simulink library "Lib_Piccolo"  (R2018b)
settings: Solver=VariableStepAuto  StartTime=0.0  StopTime=10.0  RelTol=1e-3
values from neighbouring files (symbols this model uses):
  AccelErrInt2Brakes = 0.15    [SimulationControlConfig16P.m]    (also in SimulationControlConfig16P_LEGACY.m; SimulationControlConfigTAILLESS.m = 0.2; SimulationControlConfigUTAIL.m = 0.2)
  AileronMax = 25    [SimulationControlConfig16P.m]    (also in SimulationControlConfig16P_LEGACY.m; SimulationControlConfigTAILLESS.m; SimulationControlConfigUTAIL.m)
  AileronPower = 0.00268    [SimulationControlConfig16P.m]    (also in SimulationControlConfig16P_LEGACY.m; SimulationControlConfigTAILLESS.m; SimulationControlConfigUTAIL.m)
  AileronSurfaceMax = 45    [SimulationControlConfig16P.m]    (also in SimulationControlConfig16P_LEGACY.m)
  AileronTrim = 0    [SimulationControlConfig16P.m]    (also in SimulationControlConfig16P_LEGACY.m; SimulationControlConfigTAILLESS.m; SimulationControlConfigUTAIL.m)
  Alt = 1000 + TerrainHeight    [SimulationStateConfig.m]
  AltCruise_m = testPlans(testIndx).terrainElevation * 0.3048 + 200    [SimulationControlConfig16P.m]    (also in SimulationControlConfigTAILLESS.m = 1083; SimulationControlConfigUTAIL.m = testPlans(testIndx).terrainElevation * 0.3048 + 152)
  AltitudeRate2PitchCmdIntegratorInit = 0.1    [SimulationControlPre.m]
  AltMax = 10000    [SimulationControlConfig16P.m]    (also in SimulationControlConfig16P_LEGACY.m; SimulationControlConfigTAILLESS.m; SimulationControlConfigUTAIL.m)
  AltMaxAccel = 1.25    [SimulationControlConfig16P.m]    (also in SimulationControlConfig16P_LEGACY.m = 0.9; SimulationControlConfigTAILLESS.m = 1.7; SimulationControlConfigUTAIL.m = 2)
  AltMin = 0    [SimulationControlConfig16P.m]    (also in SimulationControlConfig16P_LEGACY.m; SimulationControlConfigTAILLESS.m; SimulationControlConfigUTAIL.m)
  AltRateCmd2Pitch = 0.50    (= 0.5)    [SimulationControlConfig16P.m]    (also in SimulationControlConfig16P_LEGACY.m = 0.6; SimulationControlConfigTAILLESS.m = 0.2; SimulationControlConfigUTAIL.m = 0.3)
  AltRateError2Pitch = 0.40    (= 0.4)    [SimulationControlConfig16P.m]    (also in SimulationControlConfig16P_LEGACY.m; SimulationControlConfigTAILLESS.m = 0.55; SimulationControlConfigUTAIL.m = 0.55)
  AltRateErrorInt2Pitch = 0.50    (= 0.5)    [SimulationControlConfig16P.m]    (also in SimulationControlConfig16P_LEGACY.m = 0.45; SimulationControlConfigTAILLESS.m; SimulationControlConfigUTAIL.m = 0.75)
  AltRateLpfCutOff = 3    [SimulationControlConfig16P.m]    (also in SimulationControlConfig16P_LEGACY.m; SimulationControlConfigTAILLESS.m = 2; SimulationControlConfigUTAIL.m = 2)
  AutoNosegear2Rudder = 26    [SimulationControlConfig16P.m]    (also in SimulationControlConfig16P_LEGACY.m; SimulationControlConfigTAILLESS.m = 25.2; SimulationControlConfigUTAIL.m = 14)
  b = 5.54    [SimulationControlConfig16P.m]    (also in SimulationControlConfig16P_LEGACY.m; SimulationControlConfigTAILLESS.m = 2.37; SimulationControlConfigUTAIL.m = 2.37)
  Bank2AileronIntegratorInit = 0    [SimulationControlPre.m]
  BankMax_User = BankMax_User/180*pi    (= 0.523598775598)    [SimulationControlConfig16P.m]    (also in SimulationControlConfig16P_LEGACY.m; SimulationControlConfigTAILLESS.m = 0.610865238198; SimulationControlConfigUTAIL.m = 0.628318530718)
  baseLegFlaps = 20    [SimulationControlConfig16P.m]    (also in SimulationControlConfig16P_LEGACY.m = 0; SimulationControlConfigTAILLESS.m = 15; SimulationControlConfigUTAIL.m = 10)
  C = GeneticOpt.C    [SimulationCostFunction.m]
  c = Sw/b    (= 0.841696750903)    [SimulationControlConfig16P.m]    (also in SimulationControlConfig16P_LEGACY.m; SimulationControlConfigTAILLESS.m = 0.354008438819; SimulationControlConfigUTAIL.m = 0.354008438819)
  cell2WheelFactorMG = 5.98    [SimulationSensorConfig16P_LEGACY.m]
  cell2WheelFactorNG = 1    [SimulationSensorConfig16P_LEGACY.m]
  cellSatMaxMG = 15000    [SimulationSensorConfig16P.m]    (also in SimulationSensorConfig16P_LEGACY.m; SimulationSensorConfigTAILLESS7P.m; SimulationSensorConfigUTAIL7P.m)
  cellSatMaxNG = 1000    [SimulationSensorConfig16P.m]    (also in SimulationSensorConfig16P_LEGACY.m; SimulationSensorConfigTAILLESS7P.m; SimulationSensorConfigUTAIL7P.m)
  cellSatMinMG = -15000    [SimulationSensorConfig16P.m]    (also in SimulationSensorConfig16P_LEGACY.m; SimulationSensorConfigTAILLESS7P.m; SimulationSensorConfigUTAIL7P.m)
  cellSatMinNG = -1000    [SimulationSensorConfig16P.m]    (also in SimulationSensorConfig16P_LEGACY.m; SimulationSensorConfigTAILLESS7P.m; SimulationSensorConfigUTAIL7P.m)
  CL_Limit = CL_Max    (= 0.54)    [SimulationControlConfig16P.m]    (also in SimulationControlConfig16P_LEGACY.m; SimulationControlConfigTAILLESS.m; SimulationControlConfigUTAIL.m = 0.53)
  CL_Max = 0.54    [SimulationControlConfig16P.m]    (also in SimulationControlConfig16P_LEGACY.m; SimulationControlConfigTAILLESS.m; SimulationControlConfigUTAIL.m = 0.53)
  CL_Max_Nom = 0.465    [SimulationControlConfig16P.m]    (also in SimulationControlConfig16P_LEGACY.m; SimulationControlConfigTAILLESS.m = 0.39; SimulationControlConfigUTAIL.m)
  CL_Min = 0    [SimulationControlConfig16P.m]    (also in SimulationControlConfig16P_LEGACY.m; SimulationControlConfigTAILLESS.m; SimulationControlConfigUTAIL.m)
  ClimbMaxFraction = 0.35    [SimulationControlConfig16P.m]    (also in SimulationControlConfig16P_LEGACY.m = 0.24; SimulationControlConfigTAILLESS.m = 0.19; SimulationControlConfigUTAIL.m = 0.21)
  ClimboutMaxBank = 7.0    (= 7)    [SimulationControlConfig16P.m]    (also in SimulationControlConfig16P_LEGACY.m; SimulationControlConfigTAILLESS.m = 5; SimulationControlConfigUTAIL.m)
  ClimboutTimer = 7.0    (= 7)    [SimulationControlConfig16P.m]    (also in SimulationControlConfig16P_LEGACY.m; SimulationControlConfigTAILLESS.m; SimulationControlConfigUTAIL.m)
  dCl_per_dFlap = 0.005581818    [SimulationControlConfig16P.m]    (also in SimulationControlConfig16P_LEGACY.m = 0; SimulationControlConfigTAILLESS.m = 0; SimulationControlConfigUTAIL.m = 0)
  DecelerationCmd = 3.1    [SimulationControlConfig16P.m]    (also in SimulationControlConfig16P_LEGACY.m; SimulationControlConfigTAILLESS.m = 0.1; SimulationControlConfigUTAIL.m = 0.1)
  DeRotateLogicEndTimer = abs((NoseDownLimit_Deg-1)/DeRotateRamp_Dps)    [SimulationControlConfig16P.m]    (also in SimulationControlConfig16P_LEGACY.m; SimulationControlConfigTAILLESS.m; SimulationControlConfigUTAIL.m)
  DeRotateLogicHoldNoseUpTimer = 0.1    [SimulationControlConfig16P.m]    (also in SimulationControlConfig16P_LEGACY.m; SimulationControlConfigTAILLESS.m; SimulationControlConfigUTAIL.m)
  DeRotateLogicTimerTimeout = 2    [SimulationControlConfig16P.m]    (also in SimulationControlConfig16P_LEGACY.m; SimulationControlConfigTAILLESS.m; SimulationControlConfigUTAIL.m)
  DeRotateLowerCmdSaturation = 0    [SimulationControlConfig16P.m]    (also in SimulationControlConfig16P_LEGACY.m; SimulationControlConfigTAILLESS.m; SimulationControlConfigUTAIL.m)
  DeRotateRamp_Dps = 3    [SimulationControlConfig16P.m]    (also in SimulationControlConfig16P_LEGACY.m; SimulationControlConfigTAILLESS.m = 8; SimulationControlConfigUTAIL.m = 8)
  DeRotateUpperCmdSaturation = 7    [SimulationControlConfig16P.m]    (also in SimulationControlConfig16P_LEGACY.m; SimulationControlConfigTAILLESS.m; SimulationControlConfigUTAIL.m)
  DescentMaxFraction = 0.22    [SimulationControlConfig16P.m]    (also in SimulationControlConfig16P_LEGACY.m = 0.2; SimulationControlConfigTAILLESS.m = 0.17; SimulationControlConfigUTAIL.m = 0.17)
  DesktopSimTerrainOffset_m = 0.406    [SimulationAircraftConfig.m]
  downwindFlaps = 0    [SimulationControlConfig16P.m]    (also in SimulationControlConfig16P_LEGACY.m; SimulationControlConfigTAILLESS.m; SimulationControlConfigUTAIL.m)
  DP_init = 0.5*1.225*V_init^2    [SimulationControlConfig16P.m]    (also in SimulationControlConfig16P_LEGACY.m; SimulationControlConfigTAILLESS.m; SimulationControlConfigUTAIL.m)
  dscNoiseMG = 1    [SimulationSensorConfig16P_LEGACY.m]
  dscNoiseNG = 0.25    [SimulationSensorConfig16P_LEGACY.m]
  DSCnumBits = 24    [SimulationSensorConfig16P.m]    (also in SimulationSensorConfig16P_LEGACY.m; SimulationSensorConfigTAILLESS7P.m; SimulationSensorConfigUTAIL7P.m)
  DSCRangeMaxMG = 15000    [SimulationSensorConfig16P.m]    (also in SimulationSensorConfig16P_LEGACY.m; SimulationSensorConfigTAILLESS7P.m; SimulationSensorConfigUTAIL7P.m)
  DSCRangeMaxNG = 1000    [SimulationSensorConfig16P.m]    (also in SimulationSensorConfig16P_LEGACY.m; SimulationSensorConfigTAILLESS7P.m; SimulationSensorConfigUTAIL7P.m)
  DSCRangeMinMG = -15000    [SimulationSensorConfig16P.m]    (also in SimulationSensorConfig16P_LEGACY.m; SimulationSensorConfigTAILLESS7P.m; SimulationSensorConfigUTAIL7P.m)
  DSCRangeMinNG = -1000    [SimulationSensorConfig16P.m]    (also in SimulationSensorConfig16P_LEGACY.m; SimulationSensorConfigTAILLESS7P.m; SimulationSensorConfigUTAIL7P.m)
  dt = DLLSim.dt    [SimulationTimeStep.m]    (also in SimulationTrim.m = 0.02)
  EarlyTouchdownThreshold = 3.0    (= 3)    [SimulationControlConfig16P.m]    (also in SimulationControlConfig16P_LEGACY.m; SimulationControlConfigTAILLESS.m = 2.2; SimulationControlConfigUTAIL.m = 2.5)
  ElevatorDeflectionRate = 15    [SimulationControlConfig16P.m]    (also in SimulationControlConfig16P_LEGACY.m = 12; SimulationControlConfigTAILLESS.m = 10; SimulationControlConfigUTAIL.m = 12)
  ElevatorMax = 25    [SimulationControlConfig16P.m]    (also in SimulationControlConfig16P_LEGACY.m; SimulationControlConfigTAILLESS.m; SimulationControlConfigUTAIL.m)
  ElevatorPower = -0.002209    [SimulationControlConfig16P.m]    (also in SimulationControlConfig16P_LEGACY.m; SimulationControlConfigTAILLESS.m = -0.002956; SimulationControlConfigUTAIL.m = -0.00205983)
  ElevatorTrim = -3.5    [SimulationControlConfig16P.m]    (also in SimulationControlConfig16P_LEGACY.m; SimulationControlConfigTAILLESS.m = -6; SimulationControlConfigUTAIL.m = -8)
  elevonBias = 0    [SimulationControlConfig16P.m]    (also in SimulationControlConfig16P_LEGACY.m; SimulationControlConfigTAILLESS.m; SimulationControlConfigUTAIL.m)
  Enable_TAS_Protection = 0    [SimulationControlConfig16P.m]    (also in SimulationControlConfig16P_LEGACY.m; SimulationControlConfigTAILLESS.m; SimulationControlConfigUTAIL.m)
  EnableCrossTrackAbort = 1    [SimulationControlConfig16P.m]    (also in SimulationControlConfigTAILLESS.m; SimulationControlConfigUTAIL.m)
  EnergyBandwidth = 0.02    [SimulationControlConfig16P.m]    (also in SimulationControlConfig16P_LEGACY.m; SimulationControlConfigTAILLESS.m = 0.06; SimulationControlConfigUTAIL.m = 0.06)
  EngineLhFuelCut = 0    [SimulationAircraftConfig.m]
  EngineRhFuelCut = 0    [SimulationAircraftConfig.m]
  FastThrottleRate = 0.075    [SimulationControlConfig16P.m]    (also in SimulationControlConfig16P_LEGACY.m = 0.05; SimulationControlConfigTAILLESS.m = 0.1; SimulationControlConfigUTAIL.m = 0.1)
  FilterWarmUpTime = 2    [SimulationSensorConfig16P.m]    (also in SimulationSensorConfig16P_LEGACY.m; SimulationSensorConfigTAILLESS7P.m; SimulationSensorConfigUTAIL7P.m)
  finalApproachFlaps = 20    [SimulationControlConfig16P.m]    (also in SimulationControlConfig16P_LEGACY.m = 0; SimulationControlConfigTAILLESS.m = 22; SimulationControlConfigUTAIL.m = 10)
  FinalDescentSlope_Deg = testPlans(testIndx).descentSlope    [SimulationControlConfig16P.m]    (also in SimulationControlConfig16P_LEGACY.m; SimulationControlConfigTAILLESS.m; SimulationControlConfigUTAIL.m)
  flapMax = 0    [SimulationControlConfig16P.m]    (also in SimulationControlConfig16P_LEGACY.m; SimulationControlConfigTAILLESS.m; SimulationControlConfigUTAIL.m)
  flapRate = 7.5    [SimulationControlConfig16P.m]    (also in SimulationControlConfig16P_LEGACY.m; SimulationControlConfigTAILLESS.m = 6.6; SimulationControlConfigUTAIL.m)
  FlareHeight = 5    [SimulationControlConfig16P.m]    (also in SimulationControlConfig16P_LEGACY.m = 4.8; SimulationControlConfigTAILLESS.m = 2.5; SimulationControlConfigUTAIL.m = 2)
  FlareVerticalRate_mps = -0.4    [SimulationControlConfig16P.m]    (also in SimulationControlConfig16P_LEGACY.m = -0.5; SimulationControlConfigTAILLESS.m = -0.15; SimulationControlConfigUTAIL.m = -0.15)
  Fp_Aileron = 0.55*2*pi*RollRateLpfCutoff*dt    [SimulationControlConfig16P.m]    (also in SimulationControlConfig16P_LEGACY.m; SimulationControlConfigTAILLESS.m; SimulationControlConfigUTAIL.m)
  Fp_Alt = 0.55*AltBandwidth    (= 0.099)    [SimulationControlConfig16P.m]    (also in SimulationControlConfig16P_LEGACY.m; SimulationControlConfigTAILLESS.m = 0.587477826221; SimulationControlConfigUTAIL.m = 0.69115038379)
  Fp_AltRate = 0.55*2*pi*AltRateLpfCutOff*dt    [SimulationControlConfig16P.m]    (also in SimulationControlConfig16P_LEGACY.m; SimulationControlConfigTAILLESS.m; SimulationControlConfigUTAIL.m)
  Fp_Elevator = 0.55*2*pi*PitchRateLpfCutoff*dt    [SimulationControlConfig16P.m]    (also in SimulationControlConfig16P_LEGACY.m; SimulationControlConfigTAILLESS.m; SimulationControlConfigUTAIL.m)
  Fp_Energy = 0.55*2*pi*EnergyBandwidth    (= 0.069115038379)    [SimulationControlConfig16P.m]    (also in SimulationControlConfig16P_LEGACY.m; SimulationControlConfigTAILLESS.m = 0.207345115137; SimulationControlConfigUTAIL.m = 0.207345115137)
  Fp_Energy2 = 0.55*2*pi*EnergyBandwidth*dt    [SimulationControlConfig16P.m]    (also in SimulationControlConfig16P_LEGACY.m; SimulationControlConfigTAILLESS.m; SimulationControlConfigUTAIL.m)
  Fp_Pitch = 0.55*2*pi*PitchBandwidth    (= 2.76460153516)    [SimulationControlConfig16P.m]    (also in SimulationControlConfig16P_LEGACY.m = 3.11017672705; SimulationControlConfigTAILLESS.m = 3.80132711084; SimulationControlConfigUTAIL.m = 2.41902634326)
  Fp_Pitch_2 = 0.55*2*pi*PitchBandwidth*dt    [SimulationControlConfig16P.m]    (also in SimulationControlConfig16P_LEGACY.m; SimulationControlConfigTAILLESS.m; SimulationControlConfigUTAIL.m)
  Fp_Roll = RollBandwidth^2    (= 1)    [SimulationControlConfig16P.m]    (also in SimulationControlConfig16P_LEGACY.m = 1.44; SimulationControlConfigTAILLESS.m; SimulationControlConfigUTAIL.m)
  Fp_Rudder = 0.55*2*pi*YawRateLpfCutoff*dt    [SimulationControlConfig16P.m]    (also in SimulationControlConfig16P_LEGACY.m; SimulationControlConfigTAILLESS.m; SimulationControlConfigUTAIL.m)
  Fp_TAS = 0.55*2*pi*TASBandwidth    (= 0.103672557568)    [SimulationControlConfig16P.m]    (also in SimulationControlConfig16P_LEGACY.m; SimulationControlConfigTAILLESS.m = 0.172787595947; SimulationControlConfigUTAIL.m = 0.172787595947)
  Fp_TAS_Filter = 2*pi*TasLpfCutoff*dt    [SimulationControlConfig16P.m]    (also in SimulationControlConfig16P_LEGACY.m; SimulationControlConfigTAILLESS.m; SimulationControlConfigUTAIL.m)
  Fp_Turn = 0.55*2*pi*TurnErrLPFcutoff    (= 0.0345575191895)    [SimulationControlConfig16P.m]    (also in SimulationControlConfig16P_LEGACY.m; SimulationControlConfigTAILLESS.m = 0.172787595947; SimulationControlConfigUTAIL.m = 0.172787595947)
  Fp_TurnDerr = 0.55*2*pi*TurnDerivativeLPFcutoff    (= 0.0345575191895)    [SimulationControlConfig16P.m]    (also in SimulationControlConfig16P_LEGACY.m; SimulationControlConfigTAILLESS.m = 0.172787595947; SimulationControlConfigUTAIL.m = 0.172787595947)
  FTV = 3    [SimulationAircraftConfig.m]
  ftvStaticPositionError = 1/1.18    (= 0.847457627119)    [SimulationSensorConfig16P.m]    (also in SimulationSensorConfig16P_LEGACY.m; SimulationSensorConfigTAILLESS7P.m = 1; SimulationSensorConfigUTAIL7P.m = 1)
  g = 9.81    [SimulationStateConfig.m]
  GustSpd_Kts = testPlans(testIndx).gustSpd    [SimulationStateConfig.m]
  GustTriggerVal = testPlans(testIndx).gustTriggerVal    [SimulationStateConfig.m]
  HeadingErr2TurnRate = 0.5    [SimulationControlConfig16P.m]    (also in SimulationControlConfig16P_LEGACY.m; SimulationControlConfigTAILLESS.m; SimulationControlConfigUTAIL.m)
  HeadingErrDer2TurnRate = 0.3    [SimulationControlConfig16P.m]    (also in SimulationControlConfig16P_LEGACY.m; SimulationControlConfigTAILLESS.m; SimulationControlConfigUTAIL.m)
  IASbounce = IASstall*0.8    [SimulationControlPre.m]
  IAScruiseCMD = sqrt(2*m*9.81/(1.225*Sw*CL_cruise))    [SimulationControlConfig16P.m]    (also in SimulationControlConfig16P_LEGACY.m; SimulationControlConfigTAILLESS.m; SimulationControlConfigUTAIL.m)
  IASfinalCMD = 1.12 * IASmin    [SimulationControlConfig16P.m]    (also in SimulationControlConfig16P_LEGACY.m = 1.10 * IASmin; SimulationControlConfigTAILLESS.m = 1.10 * IASmin; SimulationControlConfigUTAIL.m = 1.15 * IASmin)
  IASflareCMD = IASstall    [SimulationControlConfig16P.m]    (also in SimulationControlConfig16P_LEGACY.m; SimulationControlConfigTAILLESS.m; SimulationControlConfigUTAIL.m)
  IASmax = 64    [SimulationControlConfig16P.m]    (also in SimulationControlConfig16P_LEGACY.m = 46; SimulationControlConfigTAILLESS.m = 38.58; SimulationControlConfigUTAIL.m = 35)
  IASmin = sqrt(2*m*9.81/(1.225*Sw*0.9*CL_Max_Nom))    [SimulationControlConfig16P.m]    (also in SimulationControlConfig16P_LEGACY.m; SimulationControlConfigTAILLESS.m; SimulationControlConfigUTAIL.m)
  IASshortCMD = IASstall    [SimulationControlConfig16P.m]    (also in SimulationControlConfig16P_LEGACY.m; SimulationControlConfigTAILLESS.m; SimulationControlConfigUTAIL.m)
  IASstall = sqrt(2*m*9.81/(1.225*Sw*CL_Max))    [SimulationControlConfig16P.m]    (also in SimulationControlConfig16P_LEGACY.m; SimulationControlConfigTAILLESS.m; SimulationControlConfigUTAIL.m)
  inFlight = 1    [SimulationControlConfig16P.m]    (also in SimulationControlConfigTAILLESS.m; SimulationControlConfigUTAIL.m)
  JetCatOffset = 5    [SimulationControlConfig16P.m]    (also in SimulationControlConfig16P_LEGACY.m)
  LaunchRollingElevator = -1.5    [SimulationControlConfig16P.m]    (also in SimulationControlConfig16P_LEGACY.m; SimulationControlConfigTAILLESS.m = 1; SimulationControlConfigUTAIL.m = 1)
  ldg_NosegearMax = 10    [SimulationControlConfig16P.m]    (also in SimulationControlConfig16P_LEGACY.m; SimulationControlConfigTAILLESS.m; SimulationControlConfigUTAIL.m)
  ldg_TrackVyErrInt2Nosegear = 0.1250    (= 0.125)    [SimulationControlConfig16P.m]    (also in SimulationControlConfig16P_LEGACY.m; SimulationControlConfigTAILLESS.m = 0.00714285714286; SimulationControlConfigUTAIL.m = 0.00714285714286)
  ldg_TrackVyErrPro2Nosegear = 0.35    [SimulationControlConfig16P.m]    (also in SimulationControlConfig16P_LEGACY.m; SimulationControlConfigTAILLESS.m = 0.0546666666667; SimulationControlConfigUTAIL.m = 0.0546666666667)
  ldg_TrackY2Vy = 0.07    [SimulationControlConfig16P.m]    (also in SimulationControlConfig16P_LEGACY.m; SimulationControlConfigTAILLESS.m = 0.17; SimulationControlConfigUTAIL.m = 0.17)
  ldg_Vy2NosegearScalingPower = 1.075    [SimulationControlConfig16P.m]    (also in SimulationControlConfig16P_LEGACY.m; SimulationControlConfigTAILLESS.m = 0.6; SimulationControlConfigUTAIL.m = 0.5)
  ldg_Y2VyScalingPower = 0.175    [SimulationControlConfig16P.m]    (also in SimulationControlConfig16P_LEGACY.m; SimulationControlConfigTAILLESS.m = 0; SimulationControlConfigUTAIL.m = 0)
  ldg_YawRate2Nosegear = 0.175    [SimulationControlConfig16P.m]    (also in SimulationControlConfig16P_LEGACY.m; SimulationControlConfigTAILLESS.m = 0.065; SimulationControlConfigUTAIL.m = 0.065)
  LiftSlope = 0.064285    [SimulationControlConfig16P.m]    (also in SimulationControlConfig16P_LEGACY.m; SimulationControlConfigTAILLESS.m = 0.058631; SimulationControlConfigUTAIL.m)
  LPFaileronInit = 0    [SimulationControlPre.m]
  LPFclestInit = 0    [SimulationControlPre.m]
  LPFenergyFFInit = 0    [SimulationControlPre.m]
  LPFtasInit = V_init + 2    [SimulationControlPre.m]
  LPFthrottleInit = ThrottleTrim    [SimulationControlPre.m]
  LPFturnErrInit = 0    [SimulationControlPre.m]
  ... (+115 more)
undefined symbols (not defined in the file or in its folder): abortFlag, alphaHPF, apmDelay, BRWNOUT, CRAWOR, CRAWUR, DiscIntNeverNeededParam, DLLSim, DLLSimStep, ECOMOR, ECOMUR, Fp_Tas, GustTrigger_HeightAgl_m, IPSTAT, LCINTEG, Ldg_Persist_Time, LOWER_FLAGS, MSG_ENABLE, NoiseStd, OLDVAL, OVERRIDE_ENABLE, OVERRIDE_VALUE, REBOOT, reversionEnable, revIASMax, revIASMin, revPitchMax, revPitchMin, revPitchRateMax, revRollMax, revRollRateMax, SAMPLE, SCALON, SensorModel, sigbuilder_block, Sim_Vx, Sim_Vy, Sim_Vz, Sim_Xpos, Sim_Ypos, Sim_Zpos, SYSOR, SYSUR, TARE, TEMPOR, TEMPUR, testIndx, testPlan, testPlans, Trim_piccoloInCmd, Trim_REFSI_FD_IN_nmodeCgShifterCmd_Ft, Trim_REFSI_FD_IN_nmodeFlapLhIBCmd_Deg, Trim_REFSI_FD_IN_nmodeFlapLhOBCmd_Deg, Trim_REFSI_FD_IN_nmodeFlapRhIBCmd_Deg, Trim_REFSI_FD_IN_nmodeFlapRhOBCmd_Deg, Trim_REFSI_FD_IN_nmodeSlatLhCmd_Deg, Trim_REFSI_FD_IN_nmodeSlatRhCmd_Deg, Trim_REFSI_FD_IN_nmodeSplrLhInbdCmd_Deg, Trim_REFSI_FD_IN_nmodeSplrLhOutbdCmd_Deg ... (+5)
libraries: simulink x866, aerolibconvert2 x60, $bdroot x52, aerolibatmos2 x5, dspswit3 x5, simulink_extras x4, dsparch4 x2, Lib_Piccolo_Alt x2, eeGeneralControl x1, dspindex x1
(part 1 of 44)
settings Model: Creator=ghoward  LastModifiedBy=JFigueira-Admin

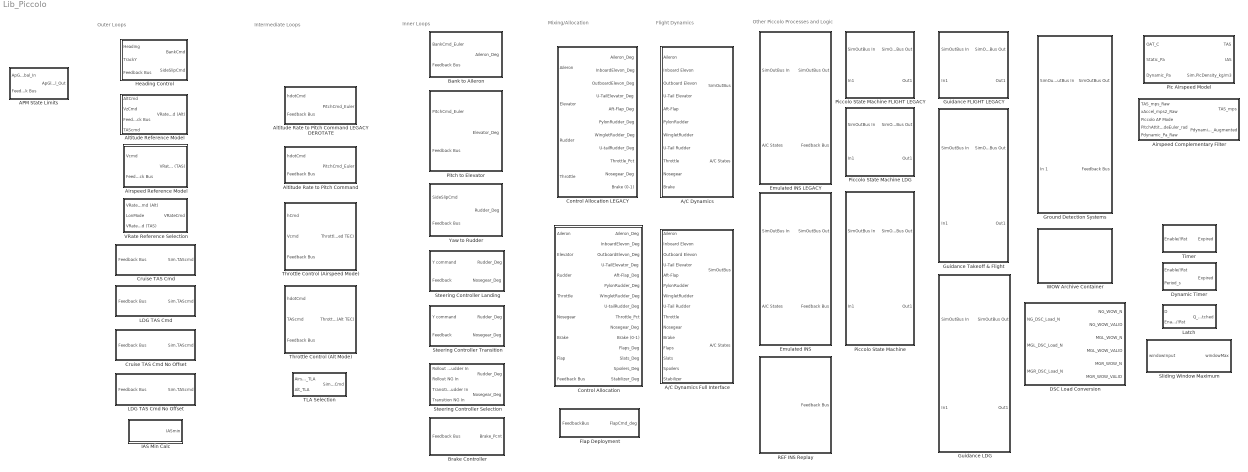
== system Lib_Piccolo ==
  note: Inner Loops
  note: Outer Loops
  note: Intermediate Loops
  note: Mixing/Allocation
  note: Other Piccolo Processes and Logic
  note: Flight Dynamics
  " Dynamic Timer" : Subsystem
      mask DialogControl DescTextVar Prompt: Timer with variable period provided as an input. Period will only be updated when reset (!RST) is active.
  " Timer" : Subsystem  mask{period=Ldg_Persist_Time}
      mask prompts: period "Period [s]"
      mask DialogControl DescGroupVar Prompt: Timer
      mask DialogControl DescTextVar Prompt: A basic timer with period as defined in mask
  A/C Dynamics : Subsystem
  A/C Dynamics Full Interface : Subsystem
  APM State Limits : Subsystem
  Airspeed Complementary Filter : Subsystem
  Airspeed Reference Model : Subsystem
  Altitude Rate to Pitch Command : Subsystem
  Altitude Rate to Pitch Command LEGACY DEROTATE : Subsystem
  Altitude Reference Model : Subsystem
  Bank to Aileron : Subsystem
  Brake Controller : Subsystem
  Control Allocation : Subsystem  Variant=on
  Control Allocation LEGACY : Subsystem
  Cruise TAS Cmd : Subsystem
  Cruise TAS Cmd No Offset : Subsystem
  DSC Load Conversion : Subsystem
  Emulated INS : Subsystem
  Emulated INS LEGACY : Subsystem
  Flap Deployment : Subsystem
  Ground Detection Systems : Subsystem
  Guidance FLIGHT LEGACY : Subsystem
  Guidance LDG : Subsystem
  Guidance Takeoff & Flight : Subsystem
  Heading Control : Subsystem
  IAS Min Calc : Subsystem
  LDG TAS Cmd : Subsystem
  LDG TAS Cmd No Offset : Subsystem
  Latch : Subsystem
  Pic Airspeed Model : Subsystem  mask{correction=1}
      mask prompts: correction "Static Position Correction"
      mask DialogControl DescGroupVar Prompt: Airspeed Indicator
      mask DialogControl DescTextVar Prompt: Model of Piccolo's Airspeed Indicator. Use 'Output Scalar' parameter to simulate errors in calculated airspeed. 'Static Position Correction' emulates behaviour of correction factor as described in PCC user's guide.
  Piccolo State Machine : Subsystem
  Piccolo State Machine FLIGHT LEGACY : Subsystem
  Piccolo State Machine LDG : Subsystem
  Pitch to Elevator : Subsystem
  REF INS Replay : Subsystem
  Sliding Window Maximum : Subsystem  mask{N=10}
      mask prompts: N "Window Size [nSamples]"
      mask DialogControl DescGroupVar Prompt: Sliding Window
      mask DialogControl DescTextVar Prompt: Sliding window (FIFO) implementation. Input sample rate and output sample rate are equal.
  Steering Controller Landing : Subsystem
  Steering Controller Selection : Subsystem
  Steering Controller Transition : Subsystem
  TLA Selection : Subsystem
  Throttle Control (Airspeed Mode) : Subsystem
  Throttle Control (Alt Mode) : Subsystem
  VRate Reference Selection : Subsystem
  WOW Archive Container : Subsystem  VariantControl=Variant
  Yaw to Rudder : Subsystem

== system Lib_Piccolo/ Dynamic Timer ==
  Enable/!Rst : Inport
  Period_s : Inport  Port=2
  Compare : RelationalOperator  OutDataTypeStr=boolean  RndMeth=Simplest
  Compare To Constant1 : simulink/Logic and Bit Operations/Compare To Constant  relop=>  const=0  OutDataTypeStr=uint8
  Compare To Constant3 : simulink/Logic and Bit Operations/Compare To Constant  relop===  const=0  OutDataTypeStr=boolean
  Discrete-Time Integrator : DiscreteIntegrator  ExternalReset=level  SampleTime=-1  OutDataTypeStr=double  ICPrevOutput=DiscIntNeverNeededParam  ICPrevScaledInput=DiscIntNeverNeededParam
  Enabled Subsystem : Subsystem  TreatAsAtomicUnit=on
  NOT : Logic  Operator=NOT  IconShape=distinctive  AllPortsSameDT=off  OutDataTypeStr=boolean
  Expired : Outport
  wires:
  Compare To Constant3/1 -> Discrete-Time Integrator/2
  Enable/!Rst/1 -> NOT/1, Compare To Constant3/1, Compare To Constant1/1  "dynamicTimer.Enable/!Rst"
  Discrete-Time Integrator/1 -> Compare/1
  Compare/1 -> Expired/1  "dynamicTimer.expired"
  Compare To Constant1/1 -> Discrete-Time Integrator/1
  Enabled Subsystem/1(periodOut) -> Compare/2  "dynamicTimer.period"
  Period_s/1 -> Enabled Subsystem/1(periodIn)
  NOT/1 -> Enabled Subsystem/Enable  "dynamicTimer.Rst/!Enable"

== system Lib_Piccolo/ Timer ==
  Enable/!Rst : Inport
  Compare To Constant1 : simulink/Logic and Bit Operations/Compare To Constant  relop=>  const=0  OutDataTypeStr=uint8
  Compare To Constant2 : simulink/Logic and Bit Operations/Compare To Constant  relop=>=  const=period  OutDataTypeStr=uint8
  Compare To Constant3 : simulink/Logic and Bit Operations/Compare To Constant  relop===  const=0  OutDataTypeStr=boolean
  Discrete-Time Integrator : DiscreteIntegrator  ExternalReset=level  SampleTime=-1  OutDataTypeStr=double  ICPrevOutput=DiscIntNeverNeededParam  ICPrevScaledInput=DiscIntNeverNeededParam
  Expired : Outport
  wires:
  Compare To Constant3/1 -> Discrete-Time Integrator/2
  Enable/!Rst/1 -> Compare To Constant3/1, Compare To Constant1/1
  Discrete-Time Integrator/1 -> Compare To Constant2/1
  Compare To Constant2/1 -> Expired/1
  Compare To Constant1/1 -> Discrete-Time Integrator/1

== system Lib_Piccolo/A//C Dynamics ==
  Aileron : Inport
  Inboard Elevon : Inport  Port=2
  Outboard Elevon : Inport  Port=3
  U-Tail Elevator : Inport  Port=4
  Aft-Flap : Inport  Port=5
  "PylonRudder " : Inport  Port=6
  WingletRudder : Inport  Port=7
  U-Tail Rudder : Inport  Port=8
  "Throttle " : Inport  Port=9
  Nosegear : Inport  Port=10
  Brake : Inport  Port=11
  Accels : Scope  Commented=on
  Airspeed : Scope  Commented=on  NumInputPorts=2
  Attitudes : Scope  Commented=on
  Bus Selector : BusSelector  Commented=on  OutputSignals=XthrustLbs,N1PctLhCmd,ismN1Lh_Pct
  Bus Selector1 : BusSelector  OutputSignals=PDps,QDps,RDps  OutputAsBus=on
  Bus Selector10 : BusSelector  OutputSignals=ZgrndNgLbs,ZgrndLhLbs,ZgrndRhLbs,GrndContactNG,GrndContactLMG,GrndContactRMG
  Bus Selector11 : BusSelector  OutputSignals=REFSI_FD_IN_nmodeAilLhUpperCmd_Deg,REFSI_FD_IN_nmodeElvLhInbdCmd_Deg,REFSI_FD_IN_nmodeElvLhOutbdCmd_Deg,REFSI_FD_IN_nmodeElvRhUTailCmd_Deg,REFSI_FD_IN_nmodeAftFlapCmd_Deg,REFSI_FD_IN_nmodeRudRhPylonCmd_Deg,REFSI_FD_IN_nmodeRudLhWingCmd_Deg,REFSI_FD_IN_nmodeRudRhUTailCmd_Deg,REFSI_FD_IN_nmodeTlaLhCmd_Deg
  Bus Selector12 : BusSelector  OutputSignals=CASKts,TASKts
  Bus Selector2 : BusSelector  Commented=on  OutputSignals=XthrustLbs,N1PctLhCmd,ismN1Lh_Pct,ismFuelBurnRateLh_Lpm,ismFuelBurntLh_Lbs  OutputAsBus=on
  Bus Selector3 : BusSelector  OutputSignals=REFSI_AC_OUT_nmodeRudLhWingCmd_Deg,REFSI_AC_OUT_nmodeAilLhLowerCmd_Deg,REFSI_AC_OUT_nmodeAilLhUpperCmd_Deg,REFSI_AC_OUT_nmodeElvLhOutbdCmd_Deg,REFSI_AC_OUT_nmodeElvLhInbdCmd_Deg,REFSI_AC_OUT_nmodeRudLhPylonCmd_Deg,REFSI_AC_OUT_nmodeRudLhUTailCmd_Deg,REFSI_AC_OUT_nmodeElvLhUTailCmd_Deg,REFSI_AC_OUT_nmodeAftFlapCmd_Deg,REFSI_AC_OUT_nmodeElvRhUTailCmd_Deg,REFSI_AC_OUT_nmodeRudRhUTailCmd_Deg,REFSI_AC_OUT_nmodeRudRhPylonCmd_Deg,REFSI_AC_OUT_nmodeElvRhInbdCmd_Deg,REFSI_AC_OUT_nmodeElvRhOutbdCmd_Deg,REFSI_AC_OUT_nmodeAilRhUpperCmd_Deg,REFSI_AC_OUT_nmodeAilRhLowerCmd_Deg,REFSI_AC_OUT_nmodeRudRhWingCmd_Deg  OutputAsBus=on
  Bus Selector4 : BusSelector  OutputSignals=PresAltFt,AlphaDeg,PDps,QDps,RDps
  Bus Selector5 : BusSelector  OutputSignals=PhiDeg,ThetaDeg,PsiDeg  OutputAsBus=on
  Bus Selector6 : BusSelector  Commented=on  OutputSignals=NxG,NyG,NzG  OutputAsBus=on
  Bus Selector7 : BusSelector  Commented=on  OutputSignals=WindUFtps,WindVFtps,WindWFtps  OutputAsBus=on
  Bus Selector8 : BusSelector  OutputSignals=XcgPctMAC  OutputAsBus=on
  Bus Selector9 : BusSelector  OutputSignals=IxxLbsInch2,IyyLbsInch2,IzzLbsInch2,IxzLbsInch2  OutputAsBus=on
  Clock : Clock
  Compare To Constant3 : simulink/Logic and Bit Operations/Compare To Constant  relop=<=  const=GustTrigger_HeightAgl_m  OutDataTypeStr=boolean
  Controls : Scope  Commented=on  NumInputPorts=9
  DLLSimulation : Subsystem
  Gain : Gain  Commented=on  Gain=1/2
  Gain1 : Gain  Commented=on  Gain=100
  Gain2 : Gain  Gain=0.01
  Goto Tag Visibility : GotoTagVisibility  GotoTag=CLAWsCommands
  Goto1 : Goto  Commented=on  GotoTag=Sim_Surface  TagVisibility=global
  Gust Wind Input1 : Subsystem  Variant=on
  Innertia : Scope  Commented=on
  Jack Fail Flags : Subsystem
  Mux : Mux
  Rates : Scope  Commented=on
  Raw Sensor Sources Alternate : Subsystem
  Raw Sensor Sources Jack : Subsystem  Commented=on
  SIM Exit Conditions : Subsystem
  Scope1 : Scope  Commented=on
  Scope2 : Scope  Commented=on  NumInputPorts=2
  Scope3 : Scope  Commented=on
  Simulated Piccolo Commands : Subsystem
  Terminator{1..11} (11 alike) : Terminator
  To Workspace : ToWorkspace  VariableName=TimeOut  SaveFormat=Structure With Time  SampleTime=-1
  To Workspace1 : ToWorkspace  Commented=on  VariableName=SimOut  SaveFormat=Timeseries  SampleTime=-1
  Unit Delay1 : UnitDelay  SampleTime=-1
  Wind : Scope  Commented=on
  lb to N : Gain  Commented=on  Gain=4.44822
  xcg : Scope  Commented=on
  SimOutBus : Outport
  A/C States : Outport  Port=2
  tag scope: CLAWsCommands=scoped
  wires:
  Bus Selector2/1 -> Bus Selector/1
  Bus Selector7/1 -> Wind/1
  Clock/1 -> To Workspace/1
  Bus Selector4/1 -> Scope3/1, Terminator1/1  "<PresAltFt>"
  Bus Selector/2 -> Scope2/1  "<N1PctLhCmd>"
  lb to N/1 -> Gain/1  "XthrustN"
  Bus Selector/1 -> lb to N/1  "<XthrustLbs>"
  Bus Selector/3 -> Gain1/1  "<ismN1Lh_Pct>"
  Gain/1 -> Scope1/1  "Simulated Results"
  Bus Selector4/5 -> Terminator5/1  "<RDps>"
  Bus Selector8/1 -> xcg/1
  Bus Selector6/1 -> Accels/1
  Bus Selector3/1 -> Unit Delay1/1
  Bus Selector9/1 -> Innertia/1
  Bus Selector12/2 -> Airspeed/2  "<TASKts>"
  Unit Delay1/1 -> [CLAWsCommands]
  Bus Selector5/1 -> Attitudes/1
  Bus Selector4/3 -> Terminator3/1  "<PDps>"
  Bus Selector4/2 -> Terminator2/1  "<AlphaDeg>"
  Gain1/1 -> Scope2/2  "ismN1Lh_Pct*100"
  Bus Selector4/4 -> Terminator4/1  "<QDps>"
  Bus Selector12/1 -> Airspeed/1  "<CASKts>"
  Bus Selector1/1 -> Rates/1
  Aileron/1 -> Simulated Piccolo Commands/1(Aileron)
  Inboard Elevon/1 -> Simulated Piccolo Commands/2(Inboard Elevon)
  Outboard Elevon/1 -> Simulated Piccolo Commands/3(Outboard Elevon)
  U-Tail Elevator/1 -> Simulated Piccolo Commands/4(U-Tail Elevator)
  "PylonRudder "/1 -> Simulated Piccolo Commands/6("PylonRudder ")
  WingletRudder/1 -> Simulated Piccolo Commands/7("WingletRudder ")
  U-Tail Rudder/1 -> Simulated Piccolo Commands/8(U-Tail Rudder)
  Bus Selector11/1 -> Mux/1, Controls/1  "<REFSI_FD_IN_nmodeAilLhUpperCmd_Deg>"
  Bus Selector11/2 -> Controls/2  "<REFSI_FD_IN_nmodeElvLhInbdCmd_Deg>"
  Bus Selector11/3 -> Controls/3  "<REFSI_FD_IN_nmodeElvLhOutbdCmd_Deg>"
  Bus Selector11/4 -> Controls/4  "<REFSI_FD_IN_nmodeElvRhUTailCmd_Deg>"
  Bus Selector11/5 -> Controls/5, Mux/2  "<REFSI_FD_IN_nmodeAftFlapCmd_Deg>"
  Bus Selector11/6 -> Controls/6, Mux/3  "<REFSI_FD_IN_nmodeRudRhPylonCmd_Deg>"
  Bus Selector11/7 -> Controls/7  "<REFSI_FD_IN_nmodeRudLhWingCmd_Deg>"
  Bus Selector11/8 -> Controls/8  "<REFSI_FD_IN_nmodeRudRhUTailCmd_Deg>"
  Bus Selector11/9 -> Gain2/1, Controls/9  "<REFSI_FD_IN_nmodeTlaLhCmd_Deg>"
  Aft-Flap/1 -> Simulated Piccolo Commands/5(Aft-Flap)
  Mux/1 -> Goto1/1
  Gain2/1 -> Mux/4
  Bus Selector10/1 -> Terminator6/1  "<ZgrndNgLbs>"
  Bus Selector10/2 -> Terminator7/1  "<ZgrndLhLbs>"
  Bus Selector10/3 -> Terminator8/1  "<ZgrndRhLbs>"
  Bus Selector10/4 -> Terminator9/1  "<GrndContactNG>"
  Bus Selector10/5 -> Terminator10/1  "<GrndContactLMG>"
  Bus Selector10/6 -> Terminator11/1  "<GrndContactRMG>"
  DLLSimulation/1(SimOutputBus) -> Jack Fail Flags/1(In1), SIM Exit Conditions/1(In1), SimOutBus/1, Raw Sensor Sources Alternate/1(In1), Raw Sensor Sources Jack/1(In1), Bus Selector5/1, Bus Selector10/1, Bus Selector12/1, Bus Selector7/1, Bus Selector6/1, Bus Selector3/1, Bus Selector2/1, Bus Selector1/1, Bus Selector4/1, Bus Selector9/1, Bus Selector8/1, To Workspace1/1
  Raw Sensor Sources Alternate/1(Out1) -> A/C States/1
  Brake/1 -> Simulated Piccolo Commands/14(Brake)
  Simulated Piccolo Commands/1(Command Bundle) -> Gust Wind Input1/1(BA Sim Input IN)
  Gust Wind Input1/1(BA Sim Input OUT) -> DLLSimulation/1(SimInputBus), Bus Selector11/1
  [AltAGL_m] -> Compare To Constant3/1
  Compare To Constant3/1 -> Gust Wind Input1/2(Trigger)
  "Throttle "/1 -> Simulated Piccolo Commands/9("Throttle ")
  Nosegear/1 -> Simulated Piccolo Commands/10(Nosegear)

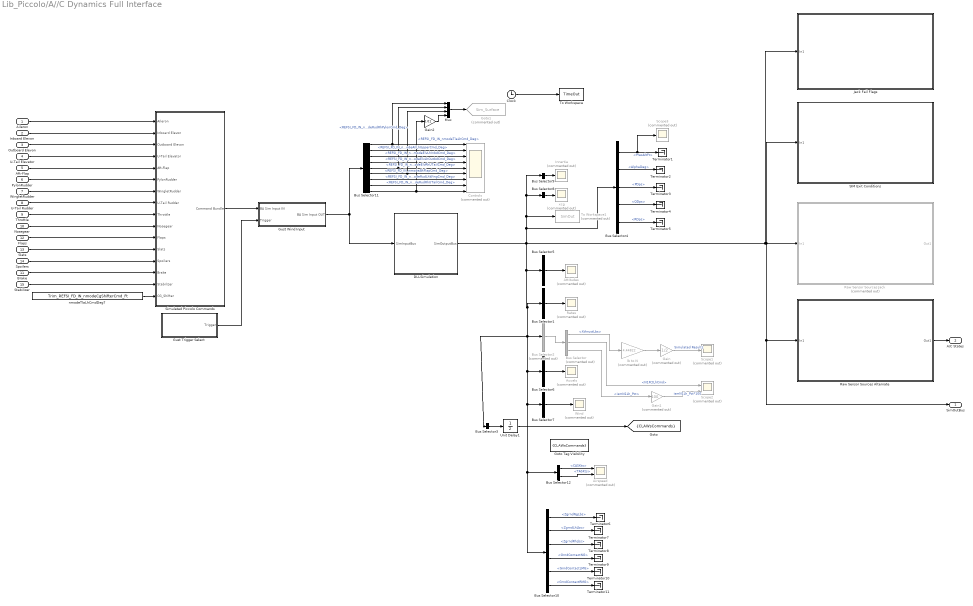
== system Lib_Piccolo/A//C Dynamics Full Interface ==
  Aileron : Inport
  Inboard Elevon : Inport  Port=2
  Outboard Elevon : Inport  Port=3
  U-Tail Elevator : Inport  Port=4
  Aft-Flap : Inport  Port=5
  "PylonRudder " : Inport  Port=6
  WingletRudder : Inport  Port=7
  U-Tail Rudder : Inport  Port=8
  "Throttle " : Inport  Port=9
  Nosegear : Inport  Port=10
  Brake : Inport  Port=11
  Flaps : Inport  Port=12
  Slats : Inport  Port=13
  Spoilers : Inport  Port=14
  Stabilizer : Inport  Port=15
  Accels : Scope  Commented=on
  Airspeed : Scope  Commented=on  NumInputPorts=2
  Attitudes : Scope  Commented=on
  Bus Selector : BusSelector  Commented=on  OutputSignals=XthrustLbs,N1PctLhCmd,ismN1Lh_Pct
  Bus Selector1 : BusSelector  OutputSignals=PDps,QDps,RDps  OutputAsBus=on
  Bus Selector10 : BusSelector  OutputSignals=ZgrndNgLbs,ZgrndLhLbs,ZgrndRhLbs,GrndContactNG,GrndContactLMG,GrndContactRMG
  Bus Selector11 : BusSelector  OutputSignals=REFSI_FD_IN_nmodeAilLhUpperCmd_Deg,REFSI_FD_IN_nmodeElvLhInbdCmd_Deg,REFSI_FD_IN_nmodeElvLhOutbdCmd_Deg,REFSI_FD_IN_nmodeElvRhUTailCmd_Deg,REFSI_FD_IN_nmodeAftFlapCmd_Deg,REFSI_FD_IN_nmodeRudRhPylonCmd_Deg,REFSI_FD_IN_nmodeRudLhWingCmd_Deg,REFSI_FD_IN_nmodeRudRhUTailCmd_Deg,REFSI_FD_IN_nmodeTlaLhCmd_Deg
  Bus Selector12 : BusSelector  OutputSignals=CASKts,TASKts
  Bus Selector2 : BusSelector  Commented=on  OutputSignals=XthrustLbs,N1PctLhCmd,ismN1Lh_Pct,ismFuelBurnRateLh_Lpm,ismFuelBurntLh_Lbs  OutputAsBus=on
  Bus Selector3 : BusSelector  OutputSignals=REFSI_AC_OUT_nmodeRudLhWingCmd_Deg,REFSI_AC_OUT_nmodeAilLhLowerCmd_Deg,REFSI_AC_OUT_nmodeAilLhUpperCmd_Deg,REFSI_AC_OUT_nmodeElvLhOutbdCmd_Deg,REFSI_AC_OUT_nmodeElvLhInbdCmd_Deg,REFSI_AC_OUT_nmodeRudLhPylonCmd_Deg,REFSI_AC_OUT_nmodeRudLhUTailCmd_Deg,REFSI_AC_OUT_nmodeElvLhUTailCmd_Deg,REFSI_AC_OUT_nmodeAftFlapCmd_Deg,REFSI_AC_OUT_nmodeElvRhUTailCmd_Deg,REFSI_AC_OUT_nmodeRudRhUTailCmd_Deg,REFSI_AC_OUT_nmodeRudRhPylonCmd_Deg,REFSI_AC_OUT_nmodeElvRhInbdCmd_Deg,REFSI_AC_OUT_nmodeElvRhOutbdCmd_Deg,REFSI_AC_OUT_nmodeAilRhUpperCmd_Deg,REFSI_AC_OUT_nmodeAilRhLowerCmd_Deg,REFSI_AC_OUT_nmodeRudRhWingCmd_Deg  OutputAsBus=on
  Bus Selector4 : BusSelector  OutputSignals=PresAltFt,AlphaDeg,PDps,QDps,RDps
  Bus Selector5 : BusSelector  OutputSignals=PhiDeg,ThetaDeg,PsiDeg  OutputAsBus=on
  Bus Selector6 : BusSelector  OutputSignals=NxG,NyG,NzG  OutputAsBus=on
  Bus Selector7 : BusSelector  OutputSignals=WindUFtps,WindVFtps,WindWFtps  OutputAsBus=on
  Bus Selector8 : BusSelector  OutputSignals=XcgPctMAC  OutputAsBus=on
  Bus Selector9 : BusSelector  OutputSignals=IxxLbsInch2,IyyLbsInch2,IzzLbsInch2,IxzLbsInch2  OutputAsBus=on
  Clock : Clock
  Controls : Scope  Commented=on  NumInputPorts=9
  DLLSimulation : Subsystem
  Gain : Gain  Commented=on  Gain=1/2
  Gain1 : Gain  Commented=on  Gain=100
  Gain2 : Gain  Gain=0.01
  Goto Tag Visibility : GotoTagVisibility  GotoTag=CLAWsCommands
  Goto1 : Goto  Commented=on  GotoTag=Sim_Surface  TagVisibility=global
  Gust Trigger Select : Subsystem  Variant=on
  Gust Wind Input : Subsystem  Variant=on
  Innertia : Scope  Commented=on
  Jack Fail Flags : Subsystem
  Mux : Mux
  Rates : Scope  Commented=on
  Raw Sensor Sources Alternate : Subsystem
  Raw Sensor Sources Jack : Subsystem  Commented=on
  SIM Exit Conditions : Subsystem
  Scope1 : Scope  Commented=on
  Scope2 : Scope  Commented=on  NumInputPorts=2
  Scope3 : Scope  Commented=on
  Simulated Piccolo Commands : Subsystem
  Terminator{1..11} (11 alike) : Terminator
  To Workspace : ToWorkspace  VariableName=TimeOut  SaveFormat=Structure With Time  SampleTime=-1
  To Workspace1 : ToWorkspace  Commented=on  VariableName=SimOut  SaveFormat=Timeseries  SampleTime=-1
  Unit Delay1 : UnitDelay  SampleTime=-1
  Wind : Scope  Commented=on
  lb to N : Gain  Commented=on  Gain=4.44822
  nmodeTlaLhCmdDeg7 : Constant  Value=Trim_REFSI_FD_IN_nmodeCgShifterCmd_Ft
  xcg : Scope  Commented=on
  SimOutBus : Outport
  A/C States : Outport  Port=2
  tag scope: CLAWsCommands=scoped
  wires:
  Gust Wind Input/1(BA Sim Input OUT) -> Bus Selector11/1, DLLSimulation/1(SimInputBus)
  Bus Selector2/1 -> Bus Selector/1
  Bus Selector7/1 -> Wind/1
  Clock/1 -> To Workspace/1
  Bus Selector4/1 -> Scope3/1, Terminator1/1  "<PresAltFt>"
  Bus Selector/2 -> Scope2/1  "<N1PctLhCmd>"
  lb to N/1 -> Gain/1
  Bus Selector/1 -> lb to N/1  "<XthrustLbs>"
  Bus Selector/3 -> Gain1/1  "<ismN1Lh_Pct>"
  Gain/1 -> Scope1/1  "Simulated Results"
  Bus Selector4/5 -> Terminator5/1  "<RDps>"
  Bus Selector8/1 -> xcg/1
  Bus Selector6/1 -> Accels/1
  Bus Selector3/1 -> Unit Delay1/1
  Bus Selector9/1 -> Innertia/1
  Bus Selector12/2 -> Airspeed/2  "<TASKts>"
  Unit Delay1/1 -> [CLAWsCommands]
  Bus Selector5/1 -> Attitudes/1
  Bus Selector4/3 -> Terminator3/1  "<PDps>"
  Bus Selector4/2 -> Terminator2/1  "<AlphaDeg>"
  Gain1/1 -> Scope2/2  "ismN1Lh_Pct*100"
  Bus Selector4/4 -> Terminator4/1  "<QDps>"
  Bus Selector12/1 -> Airspeed/1  "<CASKts>"
  Bus Selector1/1 -> Rates/1
  Bus Selector11/1 -> Mux/1, Controls/1  "<REFSI_FD_IN_nmodeAilLhUpperCmd_Deg>"
  Bus Selector11/2 -> Controls/2  "<REFSI_FD_IN_nmodeElvLhInbdCmd_Deg>"
  Bus Selector11/3 -> Controls/3  "<REFSI_FD_IN_nmodeElvLhOutbdCmd_Deg>"
  Bus Selector11/4 -> Controls/4  "<REFSI_FD_IN_nmodeElvRhUTailCmd_Deg>"
  Bus Selector11/5 -> Controls/5, Mux/2  "<REFSI_FD_IN_nmodeAftFlapCmd_Deg>"
  Bus Selector11/6 -> Controls/6, Mux/3  "<REFSI_FD_IN_nmodeRudRhPylonCmd_Deg>"
  Bus Selector11/7 -> Controls/7  "<REFSI_FD_IN_nmodeRudLhWingCmd_Deg>"
  Bus Selector11/8 -> Controls/8  "<REFSI_FD_IN_nmodeRudRhUTailCmd_Deg>"
  Bus Selector11/9 -> Gain2/1, Controls/9  "<REFSI_FD_IN_nmodeTlaLhCmd_Deg>"
  Mux/1 -> Goto1/1
  Gain2/1 -> Mux/4
  Bus Selector10/1 -> Terminator6/1  "<ZgrndNgLbs>"
  Bus Selector10/2 -> Terminator7/1  "<ZgrndLhLbs>"
  Bus Selector10/3 -> Terminator8/1  "<ZgrndRhLbs>"
  Bus Selector10/4 -> Terminator9/1  "<GrndContactNG>"
  Bus Selector10/5 -> Terminator10/1  "<GrndContactLMG>"
  Bus Selector10/6 -> Terminator11/1  "<GrndContactRMG>"
  DLLSimulation/1(SimOutputBus) -> Jack Fail Flags/1(In1), SIM Exit Conditions/1(In1), Raw Sensor Sources Alternate/1(In1), SimOutBus/1, Raw Sensor Sources Jack/1(In1), Bus Selector5/1, Bus Selector10/1, Bus Selector12/1, Bus Selector7/1, Bus Selector6/1, Bus Selector3/1, Bus Selector2/1, Bus Selector1/1, Bus Selector4/1, Bus Selector9/1, Bus Selector8/1, To Workspace1/1
  Raw Sensor Sources Alternate/1(Out1) -> A/C States/1
  Aileron/1 -> Simulated Piccolo Commands/1(Aileron)
  Aft-Flap/1 -> Simulated Piccolo Commands/5(Aft-Flap)
  WingletRudder/1 -> Simulated Piccolo Commands/7("WingletRudder ")
  Brake/1 -> Simulated Piccolo Commands/14(Brake)
  "PylonRudder "/1 -> Simulated Piccolo Commands/6("PylonRudder ")
  Simulated Piccolo Commands/1(Command Bundle) -> Gust Wind Input/1(BA Sim Input IN)
  U-Tail Rudder/1 -> Simulated Piccolo Commands/8(U-Tail Rudder)
  U-Tail Elevator/1 -> Simulated Piccolo Commands/4(U-Tail Elevator)
  Inboard Elevon/1 -> Simulated Piccolo Commands/2(Inboard Elevon)
  Stabilizer/1 -> Simulated Piccolo Commands/15(Stabilizer)
  Flaps/1 -> Simulated Piccolo Commands/11(Flaps)
  Slats/1 -> Simulated Piccolo Commands/12(Slats)
  nmodeTlaLhCmdDeg7/1 -> Simulated Piccolo Commands/16(CG_Shifter)
  Gust Trigger Select/1(Trigger) -> Gust Wind Input/2(Trigger)
  Spoilers/1 -> Simulated Piccolo Commands/13(Spoilers)
  Nosegear/1 -> Simulated Piccolo Commands/10(Nosegear)
  Outboard Elevon/1 -> Simulated Piccolo Commands/3(Outboard Elevon)
  "Throttle "/1 -> Simulated Piccolo Commands/9("Throttle ")

== system Lib_Piccolo/APM State Limits ==
  ApGlobal_In : Inport
  Feedback Bus : Inport  Port=2
  AND : Logic  Inputs=3  IconShape=distinctive  AllPortsSameDT=off  OutDataTypeStr=boolean
  Abs : Abs
  Abs1 : Abs
  Abs2 : Abs
  Bus Selector : BusSelector  OutputSignals=Roll_Euler_rad,RollRate_Body_radps,Pitch_Euler_rad,PitchRate_Body_radps,V_mps
  Clock : Clock
  Compare To Constant : simulink/Logic and Bit Operations/Compare To Constant  relop=>=  const=revRollMax  OutDataTypeStr=boolean
  Compare To Constant1 : simulink/Logic and Bit Operations/Compare To Constant  relop=>=  const=revRollRateMax  OutDataTypeStr=boolean
  Compare To Constant2 : simulink/Logic and Bit Operations/Compare To Constant  relop=>=  const=revPitchMax  OutDataTypeStr=boolean
  Compare To Constant3 : simulink/Logic and Bit Operations/Compare To Constant  relop=<=  const=revPitchMin  OutDataTypeStr=boolean
  Compare To Constant4 : simulink/Logic and Bit Operations/Compare To Constant  relop=>=  const=revPitchRateMax  OutDataTypeStr=boolean
  Compare To Constant5 : simulink/Logic and Bit Operations/Compare To Constant  relop=>=  const=revIASMax  OutDataTypeStr=boolean
  Compare To Constant6 : simulink/Logic and Bit Operations/Compare To Constant  relop=<=  const=revIASMin  OutDataTypeStr=boolean
  Compare To Constant7 : simulink/Logic and Bit Operations/Compare To Constant  relop=>  const=5  OutDataTypeStr=boolean
  Constant : Constant
  Constant1 : Constant  Value=reversionEnable
  Data Type Conversion : DataTypeConversion  OutDataTypeStr=double
  Latch : Subsystem
  OOOOOOOR : Logic  Operator=OR  Inputs=7  IconShape=distinctive  AllPortsSameDT=off  OutDataTypeStr=boolean
  Radians to Degrees{,1..3} (4 alike) : simulink_extras/Transformations/Radians to Degrees
  Switch : Switch  Criteria=u2 > Threshold  Threshold=0.5
  Terminator{,1..6} (7 alike) : Terminator
  Transport Delay : TransportDelay  DelayTime=apmDelay
  ApGlobal_Out : Outport
  wires:
  Compare To Constant7/1 -> AND/3
  Clock/1 -> Compare To Constant7/1
  ApGlobal_In/1 -> Switch/3
  Feedback Bus/1 -> Bus Selector/1
  Bus Selector/1 -> Abs/1  "<Roll_Euler_rad>"
  Bus Selector/2 -> Abs1/1  "<RollRate_Body_radps>"
  Radians to Degrees/1 -> Compare To Constant/1
  Bus Selector/3 -> Radians to Degrees2/1  "<Pitch_Euler_rad>"
  Radians to Degrees1/1 -> Compare To Constant1/1
  Radians to Degrees2/1 -> Compare To Constant3/1, Compare To Constant2/1
  Abs/1 -> Radians to Degrees/1
  Abs1/1 -> Radians to Degrees1/1
  Bus Selector/4 -> Abs2/1  "<PitchRate_Body_radps>"
  Abs2/1 -> Radians to Degrees3/1
  Bus Selector/5 -> Compare To Constant6/1, Compare To Constant5/1  "<V_mps>"
  Compare To Constant/1 -> Terminator/1, OOOOOOOR/1  "Flag_rollMax_exceeded"
  Compare To Constant1/1 -> Terminator1/1, OOOOOOOR/2  "Flag_rollRateMax_exceeded"
  Compare To Constant2/1 -> Terminator2/1, OOOOOOOR/3  "Flag_pitchMax_exceeded"
  Compare To Constant3/1 -> Terminator3/1, OOOOOOOR/4  "Flag_pitchMin_exceeded"
  Compare To Constant4/1 -> Terminator4/1, OOOOOOOR/5  "Flag_pitchRateMax_exceeded"
  Compare To Constant5/1 -> Terminator5/1, OOOOOOOR/6  "Flag_IASMax_exceeded"
  Compare To Constant6/1 -> Terminator6/1, OOOOOOOR/7  "Flag_IASMin_exceeded"
  OOOOOOOR/1 -> Data Type Conversion/1
  Constant/1 -> Latch/2(Enable/!Rst), Switch/1
  Latch/1(Q_Latched) -> Switch/2  "ReversionTriggered"
  Radians to Degrees3/1 -> Compare To Constant4/1
  AND/1 -> Latch/1(D)
  Constant1/1 -> AND/2
  Switch/1 -> ApGlobal_Out/1
  Transport Delay/1 -> AND/1
  Data Type Conversion/1 -> Transport Delay/1

== system Lib_Piccolo/Airspeed Complementary Filter ==
  TAS_mps_Raw : Inport
  xAccel_mps2_Raw : Inport  Port=2
  Piccolo AP Mode : Inport  Port=3
  PitchAttitudeEuler_rad : Inport  Port=4
  Pdynamic_Pa_Raw : Inport  Port=5
  Compare To Constant : simulink/Logic and Bit Operations/Compare To Constant  relop=>=  const=10  OutDataTypeStr=boolean
  Compare To Constant1 : simulink/Logic and Bit Operations/Compare To Constant  relop=<=  const=2  OutDataTypeStr=boolean
  Discrete-Time Integrator : DiscreteIntegrator  InitialCondition=Speed * 0.5144 + 2  SampleTime=-1  ICPrevOutput=DiscIntNeverNeededParam  ICPrevScaledInput=DiscIntNeverNeededParam
  Gain : Gain  Gain=g
  Gain1 : Gain
  Gain2 : Gain  Gain=1/2
  HPF Acceleration : Subsystem
  LPF TAS : Subsystem
  Multiply : Product
  OR : Logic  Operator=OR  IconShape=distinctive  AllPortsSameDT=off  OutDataTypeStr=boolean
  Sin : Trigonometry
  Square : Math  Operator=square  SaturateOnIntegerOverflow=on
  Sum : Sum  Inputs=+|+
  Sum1 : Sum  Inputs=|+-
  Switch : Switch  Criteria=u2 > Threshold  Threshold=0.5
  Terminator : Terminator
  TAS_mps : Outport
  Pdynamic_Pa_Augmented : Outport  Port=2
  wires:
  TAS_mps_Raw/1 -> Switch/1, LPF TAS/1(Input)
  xAccel_mps2_Raw/1 -> Sum1/1
  Compare To Constant/1 -> OR/1
  Compare To Constant1/1 -> OR/2
  OR/1 -> Switch/2  "Sim.disableTASfilter"
  Piccolo AP Mode/1 -> Compare To Constant/1, Compare To Constant1/1
  Switch/1 -> Square/1, TAS_mps/1  "REF.TAS_Filtered"
  LPF TAS/1(Output) -> Sum/1  "Sim.TAS_LPF_mps"
  Gain1/1 -> Sum/2  "Sim.HPF_AccelComponent"
  Sum/1 -> Switch/3  "Sim.Comp_TAS_mps"
  Sum1/1 -> Discrete-Time Integrator/1  "Sim.gravityCorrectedLonAccel"
  PitchAttitudeEuler_rad/1 -> Sin/1  "pitchIn"
  Sin/1 -> Gain/1
  Gain/1 -> Sum1/2
  Discrete-Time Integrator/1 -> HPF Acceleration/1(Input)  "Sim.IntegratedAccel"
  HPF Acceleration/1(Output) -> Gain1/1
  Pdynamic_Pa_Raw/1 -> Terminator/1
  Square/1 -> Multiply/1
  Gain2/1 -> Pdynamic_Pa_Augmented/1  "Sim.PdynamicAugmented"
  [PicDensity] -> Multiply/2
  Multiply/1 -> Gain2/1

== system Lib_Piccolo/Airspeed Reference Model ==
  Vcmd : Inport
  Feedback Bus : Inport  Port=2
  Airspeed Control Only Used In Airspeed Mode : Subsystem
  TAS Rate to Altitude Rate Command : Subsystem
  VRateCmd (TAS) : Outport
  wires:
  Airspeed Control Only Used In Airspeed Mode/1(VdotCmd) -> TAS Rate to Altitude Rate Command/1(VdotCmd)
  Vcmd/1 -> TAS Rate to Altitude Rate Command/3(Vcmd), Airspeed Control Only Used In Airspeed Mode/1("Vcmd ")
  TAS Rate to Altitude Rate Command/1(hdotCmd) -> VRateCmd (TAS)/1
  Feedback Bus/1 -> TAS Rate to Altitude Rate Command/2(Feedback Bus), Airspeed Control Only Used In Airspeed Mode/2(Feedback Bus)
